simulink model "sfSelfBroadcastFixed"  (R2025b)
settings: Solver=VariableStepAuto  StartTime=0.0  StopTime=10.0  RelTol=1e-3
settings Model: Creator=The MathWorks, Inc.  LastModifiedBy=The MathWorks, Inc.

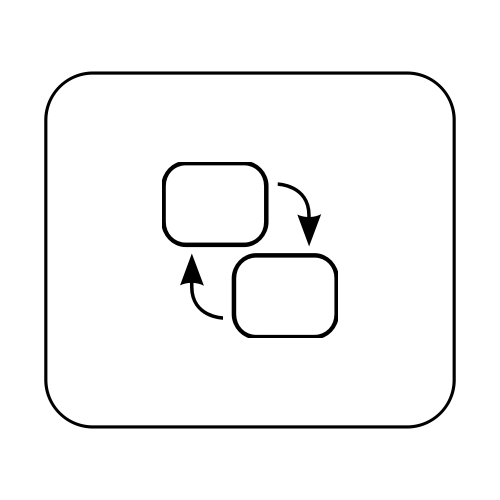
[thumbnail: Simulink's stored preview of the top-level diagram]
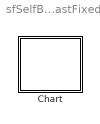
== system sfSelfBroadcastFixed ==
  Chart : Stateflow chart  TreatAsAtomicUnit=on

== stateflow chart sfSelfBroadcastFixed/Chart ==
  state A
    state B
    (default) -> B
    B -> 12
  13 -> A
